simulink model "A_SERVO_poly_shift2_u_ADAPT2_output"  (R2025b)
settings: Solver=ode15s  StartTime=0.0  StopTime=2  FixedStep=1e-5  RelTol=1e-3
values from neighbouring files (symbols this model uses):
  Ts = 0.01    [setup_nmpc.m]
  uo = [CA0s; Qs]    [setup_nmpc.m]    (also in ucompute.m = uo')
  yo = [CAs; Ts_K]    [setup_nmpc.m]    (also in ucompute.m = xo)
libraries: simulink x1
settings Model: Creator=DELL  LastModifiedBy=USER PC
settings SolverCC: AlgebraicLoopSolver=TrustRegion
settings DataIOCC: SaveFormat=StructureWithTime  ReturnWorkspaceOutputsName=cstr_out_a
settings DebuggingCC: UnconnectedInputMsg=warning  UnconnectedOutputMsg=warning  UnconnectedLineMsg=warning
settings ModelReferenceCC: EnableRefExpFcnMdlSchedulingChecks=on
settings SFSimCC: CustomCodeUndefinedFunction=UseInterfaceOnly
settings RTWCC: GPUComputeCapability=3.5

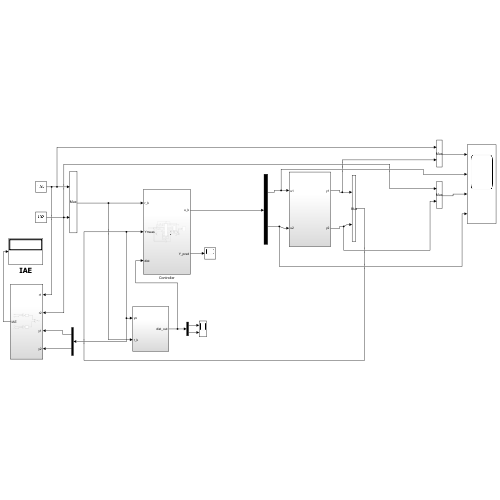
[thumbnail: Simulink's stored preview of the top-level diagram]
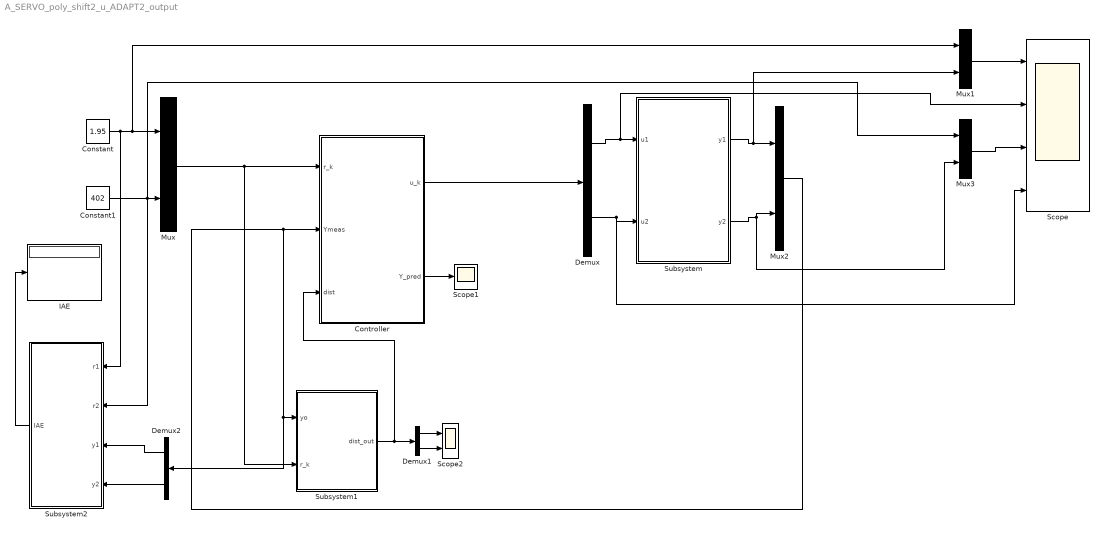
== system A_SERVO_poly_shift2_u_ADAPT2_output ==
  Constant : Constant  Value=1.95
  Constant1 : Constant  Value=402
  Controller : Subsystem
  Demux : Demux  Outputs=2
  Demux1 : Demux  Outputs=2
  Demux2 : Demux  Outputs=2
  IAE : Display
  Mux{,1..3} (4 alike) : Mux  Inputs=2
  Scope : Scope  NumInputPorts=4
      settings: SampleTime=1e-4  ActiveDisplayYMinimum=0.785141160048574  ActiveDisplayYMaximum=2.433729559562833  DataLoggingVariableName=x_data_a
  Scope1 : Scope
      settings: ActiveDisplayYMinimum=-61.83399  ActiveDisplayYMaximum=559.61994  DataLoggingVariableName=ScopeData2
  Scope2 : Scope  NumInputPorts=2
      settings: SampleTime=1e-4  ActiveDisplayYMinimum=-0.30896683359711319  ActiveDisplayYMaximum=0.18016585420133263  DataLoggingVariableName=d_data
  Subsystem : Subsystem
  Subsystem1 : Subsystem
  Subsystem2 : Subsystem
  wires:
  Controller/1(u_k) -> Demux/1
  Mux/1 -> Subsystem1/2(r_k), Controller/1(r_k)
  Mux2/1 -> Subsystem1/1(yo), Demux2/1, Controller/2(Ymeas)
  Demux/1 -> Scope/2, Subsystem/1(u1)
  Demux/2 -> Subsystem/2(u2), Scope/4
  Constant1/1 -> Subsystem2/2(r2), Mux3/1, Mux/2
  Constant/1 -> Subsystem2/1(r1), Mux1/1, Mux/1
  Subsystem/1(y1) -> Mux1/2, Mux2/1
  Subsystem/2(y2) -> Mux3/2, Mux2/2
  Mux1/1 -> Scope/1
  Mux3/1 -> Scope/3
  Controller/2(Y_pred) -> Scope1/1
  Subsystem1/1(dist_out) -> Demux1/1, Controller/3(dist)
  Demux1/1 -> Scope2/1
  Demux1/2 -> Scope2/2
  Subsystem2/1(IAE) -> IAE/1
  Demux2/1 -> Subsystem2/3(y1)
  Demux2/2 -> Subsystem2/4(y2)

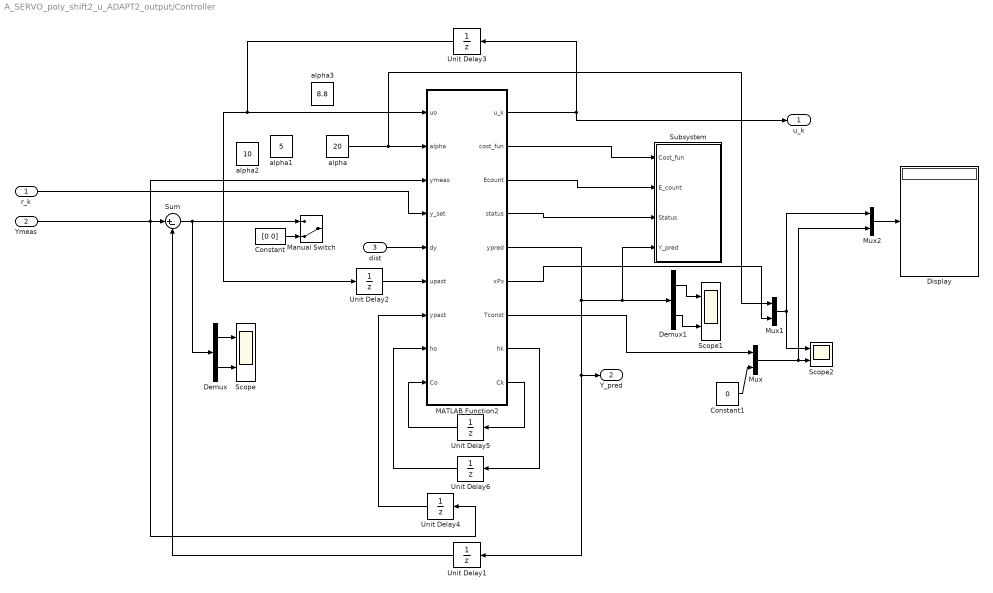
== system A_SERVO_poly_shift2_u_ADAPT2_output/Controller ==
  r_k : Inport
  Ymeas : Inport  Port=2
  dist : Inport  Port=3
  Constant : Constant  Value=[0 0]
  Constant1 : Constant  Value=0
  Demux : Demux  Outputs=2
  Demux1 : Demux  Outputs=2
  Display : Display
  MATLAB Function2 : MATLAB Function  TreatAsAtomicUnit=on
  Manual Switch : ManualSwitch  CurrentSetting=0
  Mux : Mux  Inputs=2
  Mux1 : Mux  Inputs=2
  Mux2 : Mux  Inputs=2
  Scope : Scope  NumInputPorts=2
      settings: ActiveDisplayYMinimum=-1.38424  ActiveDisplayYMaximum=0.86048
  Scope1 : Scope  NumInputPorts=2
      settings: ActiveDisplayYMinimum=0.05583  ActiveDisplayYMaximum=2.20226  DataLoggingVariableName=ScopeData3
  Scope2 : Scope  NumInputPorts=2
      settings: SampleTime=1e-4  ActiveDisplayYMinimum=-7.3315097922992862  ActiveDisplayYMaximum=8.4581074793252533  DataLoggingVariableName=Terminal_a
  Subsystem : Subsystem
  Sum : Sum  Inputs=|+-
  Unit Delay1 : UnitDelay  InitialCondition=yo  SampleTime=Ts  HasFrameUpgradeWarning=on
  Unit Delay2 : UnitDelay  InitialCondition=uo  SampleTime=Ts  HasFrameUpgradeWarning=on
  Unit Delay3 : UnitDelay  InitialCondition=uo  SampleTime=Ts  HasFrameUpgradeWarning=on
  Unit Delay4 : UnitDelay  InitialCondition=yo  SampleTime=Ts  HasFrameUpgradeWarning=on
  Unit Delay5 : UnitDelay  InitialCondition=zeros(10,1)  SampleTime=Ts  HasFrameUpgradeWarning=on
  Unit Delay6 : UnitDelay  InitialCondition=zeros(10,1)  SampleTime=Ts  HasFrameUpgradeWarning=on
  alpha : Constant  Value=20
  alpha1 : Constant  Value=5
  alpha2 : Constant  Value=10
  alpha3 : Constant  Value=8.8
  u_k : Outport  VectorParamsAs1DForOutWhenUnconnected=off
  Y_pred : Outport  Port=2  VectorParamsAs1DForOutWhenUnconnected=off
  wires:
  MATLAB Function2/4(status) -> Subsystem/3(Status)
  MATLAB Function2/3(Ecount) -> Subsystem/2(E_count)
  Unit Delay1/1 -> Sum/2
  MATLAB Function2/2(cost_fun) -> Subsystem/1(Cost_fun)
  r_k/1 -> MATLAB Function2/4(y_set)
  MATLAB Function2/1(u_k) -> u_k/1, Unit Delay3/1
  MATLAB Function2/5(ypred) -> Unit Delay1/1, Y_pred/1, Subsystem/4(Y_pred), Demux1/1
  Ymeas/1 -> Unit Delay4/1, MATLAB Function2/3(ymeas), Sum/1
  Sum/1 -> Demux/1, Manual Switch/1
  Constant/1 -> Manual Switch/2
  Unit Delay3/1 -> Unit Delay2/1, MATLAB Function2/1(uo)
  Unit Delay2/1 -> MATLAB Function2/6(upast)
  Demux/2 -> Scope/2
  Demux/1 -> Scope/1
  Demux1/1 -> Scope1/1
  Demux1/2 -> Scope1/2
  Unit Delay4/1 -> MATLAB Function2/7(ypast)
  MATLAB Function2/9(Ck) -> Unit Delay5/1
  MATLAB Function2/8(hk) -> Unit Delay6/1
  Unit Delay5/1 -> MATLAB Function2/9(Co)
  Unit Delay6/1 -> MATLAB Function2/8(ho)
  Constant1/1 -> Mux/2
  MATLAB Function2/7(Tconst) -> Mux/1
  Mux/1 -> Mux2/2, Scope2/2
  Mux1/1 -> Mux2/1, Scope2/1
  alpha/1 -> MATLAB Function2/2(alpha), Mux1/1
  MATLAB Function2/6(xPx) -> Mux1/2
  Mux2/1 -> Display/1
  dist/1 -> MATLAB Function2/5(dy)

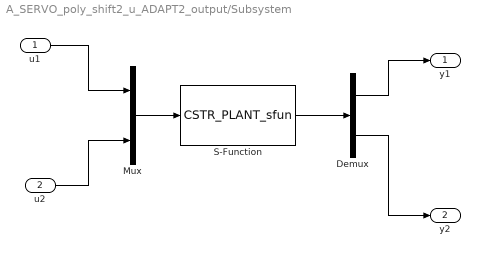
== system A_SERVO_poly_shift2_u_ADAPT2_output/Subsystem ==
  u1 : Inport
  u2 : Inport  Port=2
  Demux : Demux  Outputs=2
  Mux : Mux  Inputs=2
  S-Function : S-Function  FunctionName=CSTR_PLANT_sfun  SFunctionDeploymentMode=off  EnableBusSupport=off
  y1 : Outport
  y2 : Outport  Port=2
  wires:
  Mux/1 -> S-Function/1
  S-Function/1 -> Demux/1
  u1/1 -> Mux/1
  u2/1 -> Mux/2
  Demux/1 -> y1/1
  Demux/2 -> y2/1

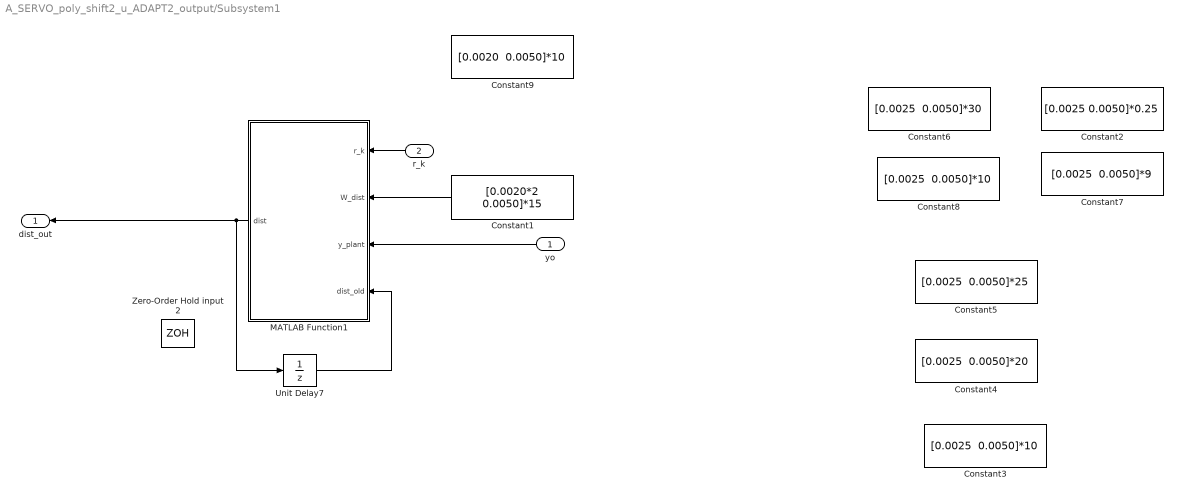
== system A_SERVO_poly_shift2_u_ADAPT2_output/Subsystem1 ==
  yo : Inport
  r_k : Inport  Port=2
  Constant1 : Constant  Value="[0.0020*2  0.0050]*15"
  Constant2 : Constant  Value="[0.0025  0.0050]*0.25"
  Constant3 : Constant  Value="[0.0025  0.0050]*10"
  Constant4 : Constant  Value="[0.0025  0.0050]*20"
  Constant5 : Constant  Value="[0.0025  0.0050]*25"
  Constant6 : Constant  Value="[0.0025  0.0050]*30"
  Constant7 : Constant  Value="[0.0025  0.0050]*9"
  Constant8 : Constant  Value="[0.0025  0.0050]*10"
  Constant9 : Constant  Value="[0.0020  0.0050]*10"
  MATLAB Function1 : MATLAB Function  TreatAsAtomicUnit=on
  Unit Delay7 : UnitDelay  InitialCondition=[0 ; 0]  SampleTime=Ts  HasFrameUpgradeWarning=on
  Zero-Order Hold input 2 : ZeroOrderHold  SampleTime=Ts/100
  dist_out : Outport  VectorParamsAs1DForOutWhenUnconnected=off
  wires:
  MATLAB Function1/1(dist) -> dist_out/1, Unit Delay7/1
  r_k/1 -> MATLAB Function1/1(r_k)
  Unit Delay7/1 -> MATLAB Function1/4(dist_old)
  Constant1/1 -> MATLAB Function1/2(W_dist)
  yo/1 -> MATLAB Function1/3(y_plant)

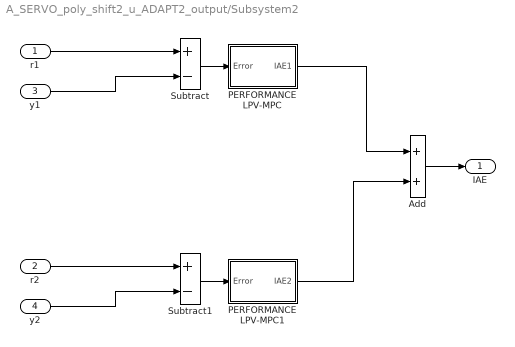
== system A_SERVO_poly_shift2_u_ADAPT2_output/Subsystem2 ==
  r1 : Inport
  r2 : Inport  Port=2
  y1 : Inport  Port=3
  y2 : Inport  Port=4
  Add : Sum
  PERFORMANCE LPV-MPC : Subsystem
  PERFORMANCE LPV-MPC1 : Subsystem
  Subtract : Sum  Inputs=+-
  Subtract1 : Sum  Inputs=+-
  IAE : Outport
  wires:
  Subtract/1 -> PERFORMANCE LPV-MPC/1(Error)
  r1/1 -> Subtract/1
  y1/1 -> Subtract/2
  y2/1 -> Subtract1/2
  r2/1 -> Subtract1/1
  Subtract1/1 -> PERFORMANCE LPV-MPC1/1(Error)
  PERFORMANCE LPV-MPC/1(IAE1) -> Add/1
  PERFORMANCE LPV-MPC1/1(IAE2) -> Add/2
  Add/1 -> IAE/1

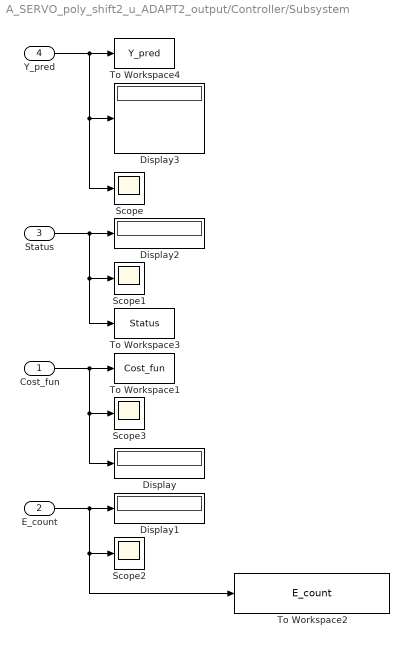
== system A_SERVO_poly_shift2_u_ADAPT2_output/Controller/Subsystem ==
  Cost_fun : Inport
  E_count : Inport  Port=2
  Status : Inport  Port=3
  Y_pred : Inport  Port=4
  Display{,1..3} (4 alike) : Display
  Scope{,1..3} (4 alike) : Scope
      Scope settings: ActiveDisplayYMinimum=-61.83399  ActiveDisplayYMaximum=559.61994  DataLoggingVariableName=ScopeData7
      Scope1 settings: ActiveDisplayYMinimum=-2.5  ActiveDisplayYMaximum=2.5  DataLoggingVariableName=ScopeData8
      Scope2 settings: ActiveDisplayYMinimum=0.50524  ActiveDisplayYMaximum=3.77769  DataLoggingVariableName=ScopeData9
      Scope3 settings: ActiveDisplayYMinimum=-35.52311  ActiveDisplayYMaximum=347.14347  DataLoggingVariableName=ScopeData10
  To Workspace1 : ToWorkspace  VariableName=Cost_fun  SaveFormat=Structure With Time  SampleTime=Ts
  To Workspace2 : ToWorkspace  VariableName=E_count  SaveFormat=Structure With Time  SampleTime=Ts
  To Workspace3 : ToWorkspace  VariableName=Status  SaveFormat=Structure With Time  SampleTime=Ts
  To Workspace4 : ToWorkspace  VariableName=Y_pred  SaveFormat=Structure With Time  SampleTime=Ts
  wires:
  Status/1 -> Scope1/1, To Workspace3/1, Display2/1
  Y_pred/1 -> Display3/1, Scope/1, To Workspace4/1
  Cost_fun/1 -> Display/1, Scope3/1, To Workspace1/1
  E_count/1 -> Scope2/1, To Workspace2/1, Display1/1

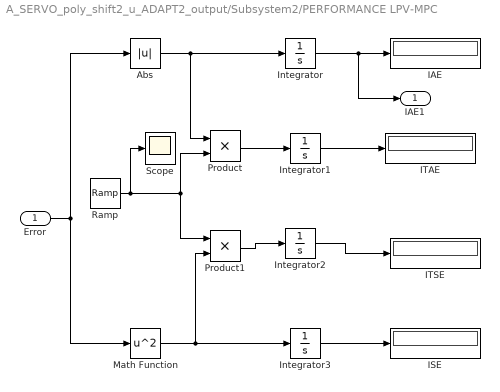
== system A_SERVO_poly_shift2_u_ADAPT2_output/Subsystem2/PERFORMANCE LPV-MPC ==
  Error : Inport
  Abs : Abs  SaturateOnIntegerOverflow=off
  IAE : Display
  ISE : Display
  ITAE : Display
  ITSE : Display
  Integrator{,1..3} (4 alike) : Integrator
  Math Function : Math  Operator=square  SignedPower=on
  Product : Product  RndMeth=Zero
  Product1 : Product  RndMeth=Zero
  Ramp : simulink/Sources/Ramp  slope=1  start=0  InitialOutput=0
  Scope : Scope
      settings: DataLoggingSaveFormat=Array
  IAE1 : Outport
  wires:
  Error/1 -> Math Function/1, Abs/1
  Abs/1 -> Integrator/1, Product/1
  Integrator/1 -> IAE1/1, IAE/1
  Ramp/1 -> Product/2, Product1/1, Scope/1
  Math Function/1 -> Integrator3/1, Product1/2
  Product1/1 -> Integrator2/1
  Product/1 -> Integrator1/1
  Integrator3/1 -> ISE/1
  Integrator2/1 -> ITSE/1
  Integrator1/1 -> ITAE/1

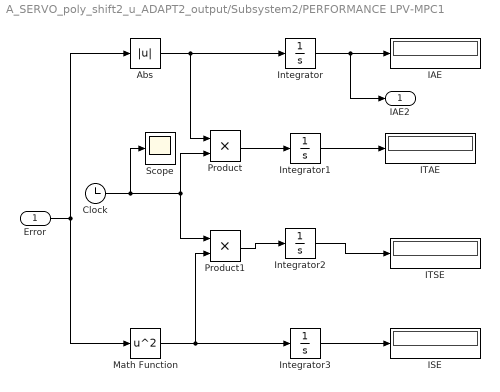
== system A_SERVO_poly_shift2_u_ADAPT2_output/Subsystem2/PERFORMANCE LPV-MPC1 ==
  Error : Inport
  Abs : Abs  SaturateOnIntegerOverflow=off
  Clock : Clock
  IAE : Display
  ISE : Display
  ITAE : Display
  ITSE : Display
  Integrator{,1..3} (4 alike) : Integrator
  Math Function : Math  Operator=square  SignedPower=on
  Product : Product  RndMeth=Zero
  Product1 : Product  RndMeth=Zero
  Scope : Scope
      settings: DataLoggingSaveFormat=Array
  IAE2 : Outport
  wires:
  Integrator1/1 -> ITAE/1
  Integrator2/1 -> ITSE/1
  Integrator3/1 -> ISE/1
  Product/1 -> Integrator1/1
  Product1/1 -> Integrator2/1
  Math Function/1 -> Product1/2, Integrator3/1
  Clock/1 -> Scope/1, Product1/1, Product/2
  Integrator/1 -> IAE2/1, IAE/1
  Abs/1 -> Product/1, Integrator/1
  Error/1 -> Abs/1, Math Function/1

== matlab function A_SERVO_poly_shift2_u_ADAPT2_output/Controller/MATLAB Function2 ==
  settings: updateMethod=DISCRETE  sampleTime=Ts
  data: uo input; alpha input; ymeas input; y_set input; dy input; upast input; u_k output; cost_fun output size=1; Ecount output; status output; ypred output; xPx output; Tconst output; ypast input; ho input; Co input; hk output; Ck output
function [u_k,cost_fun,Ecount,status,ypred,xPx, Tconst,hk,Ck] = NMPC_FT(uo,alpha,ymeas,y_set,dy,upast,ypast,ho,Co)

%#codegen
coder.extrinsic('ucompute_PINN')

r1=y_set(1)  ; 
r2=y_set(2)  ; 
 

xo=ymeas  ;



%MPC TUNNING PARAMETERS
Np=10;    % 30
Nu=2;

% Wy1=500;         Wy2=0.5;
% Wu1=1.5;           Wu2=1e-5;    
% % Wu1=0;           Wu2=0;                        
% Wdu1=18;         Wdu2=1e-5;    



% Q=diag([1/1.95 ,1/402]*10) ;
% R=diag([1/4,1e-10]*4) ;



Q=diag([1/1.95 ,1/402]*2) ;
R=diag([1/4,1e-10]) ;


Wy1=Q(1,1);         Wy2=Q(2,2);
% Wu1=R(1,1);         Wu2=R(2,2);    
Wu1=0;           Wu2=0;                        
Wdu1=R(1,1);         Wdu2=R(2,2);    

K = [0.000019585478721   0.000000223009726
   1.379183649900090   0.049533378348744 ]*1.0e+05 ;


% P = [18.678807460745315   0.509902088166268
%    0.509902088166268   0.033835699074817 ] ;

% P = [18.678807460745315   0.509902088166268
%      0.509902088166268   0.033835699074817 ] ;
P=[1060,  22 ;
   22,   0.52] ;

% K = [2.0894     0.021215
%    1.5151e+05       5683.9] ;
% 
% 
% P = [ 82.057       2.2952
%        2.2952      0.16119 ] ;




% P=[1060,  22 ;
%  22,   0.52] ;   %  P=10    P=eye(20)


% K =[4.1791    0.2335
%     5.3039   19.6972] ;
%%%%%%%%%%%%%%%%%%%%%%%%%%%%%%%%%%%%%%%%%%%%%%%%%%%%%%%%%%%%%%%%%%%%%%%%

% P = [1.3754   -0.0195
%    -0.0195    0.0104]*1000 ;

% P=[1060,  22 ;
%    22,   0.52] ;   

%%%%%%%%%%%%%%%%%%%%%%%%%%%%%%%%%%%%%%%%%%%%%%%%%%%%%%%%%%%%%%%%%%%%%%%%
% rhomin=2 ;


% K =[1.4724    0.0736
%   306.2690   33.8670 ] ;
% 
% 
% P =[2.8131    0.0643
%     0.0643    0.0146]*1000  ;

% K =[0.0001   -0.0000
%     1.4005    0.3482]*1.0e+05 ;
% 
% 
% P =[719.3780   -7.4821
%    -7.4821    0.9092] ;



% K =[4.4232    0.2320
%    44.8060   21.0231] ;
% 
% 
% P =[1.3256   -0.0084
%    -0.0084    0.0110]*1000;



% K =[3.4260    0.1780
%    89.6741   23.3041];
% 
% 
% P =[1.5757    0.0042
%     0.0042    0.0117]*1000 ;



% Wy1=1/3.15;         Wy2=1/344;         
% Wu1=0;           Wu2=0;                        
% Wdu1=1/3.5;        Wdu2=1/340;   

% Wy1=1/3.15;         Wy2=1/344;         
% Wu1=0;              Wu2=0;                        
% Wdu1=1/3.5*10;      Wdu2=1/340*10;  



% SAMPLING TIME FOR DISCRETIZATION

%%%%%%%%%%%%%%%%%%%%%%%%%%
% PROCESS CONSTRAINTS ON Y, U AND DELTA_U
%%%%%%%%%%%%%%%%%%%%%%%%%%
% PROCESS CONSTRAINTS ON Y, U AND DELTA_U
% ManipulatedVariables(1)=struct('Min',2,'Max',5,'RateMin',-xM,'Ratemax',xM,'Units','per_min')
% ManipulatedVariables(2)=struct('Min',326,'Max',360,'RateMin',-xT,'Ratemax',xT,'Units','per_min')
% 
% OutputVariables(1)=struct('Min',0,'Max',5,'Units','per_min')
% OutputVariables(2)=struct('Min',0,'Max',360,'Units','per_min')

x1min=0.6;     x2min=0;        
x1max=5;     x2max=600;      


u1min=0.5;      u2min=-5e5;        
u1max=7.5;     u2max=5e5;      

du1min=-3.5;   du2min=-5e5;  
du1max=3.5;    du2max=5e5;   


UMIN_colvector=[u1min*ones(Nu,1);u2min*ones(Nu,1)];
UMAX_colvector=[u1max*ones(Nu,1);u2max*ones(Nu,1)];



%%%%%%%%%%%%%%%%%%%%%%%%%%%%%%%%%%%%%%%%%%%%%%%
% PROCESS INPUT TRAJECTORY

% uo=[3.5 ; 340] ;
% yo=[3.149;344.1] ;
% Ts=180 ;

u1set=4  ;
u2set=0   ;


%%%%%%%%%%%%%%%%%%%%%%%%%%%%%%%%%%%%%%%%%%%%%%%
% STARTING POINT FOR THE OPTIMIZATION ALGORITHM

uo_start=[4 ; 1e-4] ;

U_initial=[uo_start(1)*ones(Nu,1);uo_start(2)*ones(Nu,1)];
 
%%%%%%%%%%%%%%%%%%%%%%%%


u_first_move = [0;0]  ;
fcost = inf  ;
ypred =[0;0]  ;
Ecount = 0  ;
exitflag = 2;
hk=zeros(10,1);
Ck=zeros(10,1);
xPx=0 ;
Tconst=0;



% [u_first_move,fcost,Ecount,exitflag,ypred,hk,Ck,xPx, Tconst]=ucompute(r1,r2,u1set,u2set,Wy1,Wy2...
%     ,Wu1,Wu2,Wdu1,Wdu2,xo,uo,upast,ypast,Np,Nu,dy...
%     ,x1min,x2min,x1max,x2max,du1min,du2min,du1max,du2max...
%     ,U_initial,UMIN_colvector,UMAX_colvector,ho,Co,P,alpha) ;

[u_first_move,fcost,Ecount,exitflag,ypred,hk,Ck,xPx, Tconst]=ucompute_PINN(r1,r2,u1set,u2set,Wy1,Wy2...
    ,Wu1,Wu2,Wdu1,Wdu2,xo,uo,upast,ypast,Np,Nu,dy...
    ,x1min,x2min,x1max,x2max,du1min,du2min,du1max,du2max...
    ,U_initial,UMIN_colvector,UMAX_colvector,ho,Co,P,alpha) ;



u_k=u_first_move  ;


status = exitflag;
cost_fun=fcost  ;

== matlab function A_SERVO_poly_shift2_u_ADAPT2_output/Subsystem1/MATLAB Function1 ==
  data: r_k input size=[2,1]; W_dist input; y_plant input size=[2,1]; dist_old input; dist output size=[2,1]
function dist = Dist_rejector(r_k,W_dist,y_plant,dist_old)
%This simply compares the plant output with the predicted output and
%calculates the difference
e_k = y_plant - r_k;

% error_min = -10; %Minimum permissible error
% error_max = +10; %Maximum permissible error

error_min = -200; %Minimum permissible error
error_max = +200; %Maximum permissible error


error_func = zeros(2,1);
dist = zeros(2,1);

if e_k(1) > error_min && e_k(1) < error_max 
    % error_func(1) = tanh(e_k(1));
    error_func(1) = (e_k(1));
else
    error_func(1) = 0;
end

if e_k(2) > error_min && e_k(2) < error_max 
    % error_func(2) = tanh(e_k(2));
    error_func(2) = (e_k(2));
else
    error_func(2) = 0;
end


%The disturbance function is a linear function of the error function.

dist(1) = (error_func(1)*W_dist(1)) + dist_old(1);
dist(2) = (error_func(2)*W_dist(2)) + dist_old(2);
